simulink model "EV6_LUT_FourWheel_EV6Battery77p4kWh_PowerCorrected"  (R2024a)
settings: Solver=ode4  StartTime=0  StopTime=60  FixedStep=0.001  RelTol=1e-3
PreLoadFcn:
  | VSS_BICYCLE=Simulink.Variant('Dual=0');
  | VSS_DUAL=Simulink.Variant('Dual=1');
  | Dual=1;
  | load('DriveCycle2.mat')
PostLoadFcn:
  | if any(exist('dsrtsu_mdlpostloadfcn', 'file') ~= 0), dsrtsu_mdlpostloadfcn('Execute', bdroot); end
InitFcn:
  | , if any(exist('rtifpga_mdlclblib', 'file') ~= 0), rtifpga_mdlclblib('Init', bdroot); end,
  | , if any(exist('dsmpb_private', 'file') ~= 0), dsmpb_private('dsmpb_mdlclblib', 'Init', bdroot); end,
  | load('DriveCycle2.mat')
model workspace (MAT data in the model file):
  DiffRatio = 10.65
  EV6_2023_BattBranchCapacity_Ah = 55.5236728838
  EV6_2023_BattEnergy_kWh = 77.4
  EV6_2023_BattNominalVoltage_V = 697
  EV6_2023_BattNumCellsParallel = 2
  EV6_2023_BattNumCellsSeries = 192
  EV6_2023_BattOpenVoltCapBpts = [0 0.1 0.2 0.3 0.4 0.5 0.6 0.7 0.8 0.9 1]
  EV6_2023_BattOpenVoltTbl = [2.96762142548 3.40364281191 3.47417488548 3.54470541822 3.61523441014 3.68576186124 3.75628777151 3.82681214095 3.94527005036 4.07101207308 4.2120755254]
  EV6_2023_BattPackCapacity_Ah = 111.047345768
  EV6_2023_BattResistSocBpts = [0 0.2 0.4 0.6 0.8 1]
  EV6_2023_BattResistTbl = [0.0163620057716 0.0118174152018 0.00807187352333 0.00375663957972 0.00266904525531 0.00103635901355 0.0019014404175 0.0172368903217 0.0121226074867 0.00758541551769 0.00474065349228 0.00337561163613 ... (42 elements, 7x6)]
  EV6_2023_BattResistTempBpts = [243.1 253.1 263.1 273.1 283.1 298.1 313.1]
  EV6_2023_InitialPackOCV_V = 726.471714233
  EV6_2023_InitialSOC = 0.638878863672
  EV6_BattCellCapacity_Ah = 60.3
  EV6_BattInitialSOC = 0.638878863672
  EV6_BattOCV_Cell_V = [2.96762142548 3.40364281191 3.47417488548 3.54470541822 3.61523441014 3.68576186124 3.75628777151 3.82681214095 3.94527005036 4.07101207308 4.2120755254]
  EV6_BattOCV_SOC = [0 0.1 0.2 0.3 0.4 0.5 0.6 0.7 0.8 0.9 1]
  EV6_BattPackCapacity_Ah = 120.6
  EV6_BattParallelCells = 2
  EV6_BattResistanceSOC = [0 0.2 0.4 0.6 0.8 1]
  EV6_BattResistanceTable_Ohm = [0.0163620057716 0.0118174152018 0.00807187352333 0.00375663957972 0.00266904525531 0.00103635901355 0.0019014404175 0.0172368903217 0.0121226074867 0.00758541551769 0.00474065349228 0.00337561163613 ... (42 elements, 7x6)]
  EV6_BattResistanceTemp_K = [243.1 253.1 263.1 273.1 283.1 298.1 313.1]
  EV6_BattSeriesCells = 192
  EV6_FinalDriveRatio = 10.65
  EV6_TargetPackResistance_Ohm = 0.132763804608
  Gas = 0.383333333333
undefined symbols (not defined in the file): accel_bp_mps2, AccelCmd, ActTqLF_Nm_, ActTqLR_Nm_, ActTqRF_Nm_, ActTqRR_Nm_, BattChargeLimitMaxPwr, BattChargeLimitSocBpts, BattChargeLimitTbl, BattDischargeLimitSocBpts, BattDischargeLimitTbl, BattDischargeMaxPwr, BrakeMaxPrs, BrakeMaxTrq, ChassisDistCg2FrontAxle, ChassisDistCg2RearAxle, ChassisVehMass, CltchCmd, CoastDown, DecelCmd, DiscIntNeverNeededParam, EnvGravCnst, EnvPrs, EnvTemp, EV6_RegenTorqueGain, EV6_TractionTorqueGain, front_share_regen_3d, front_share_traction_3d, FuelSpecificGrav, GearCmd, h, InitStates, lgSw, limitedMCT, MCT, MtrEffSpdBpts, MtrEffTbl, MtrEffTrqBpts, MtrPwrMax, MtrTrqMax, out_1, pMCT, RealSimPara, Ref_speed, Ref_time, regen_torque_bp_Nm, speed_bp_kph, SteeringCmd, SupvsryCtrlRegenBrkCutOffTbl, SupvsryCtrlRegenSpdBpts, TestScnrioCycleNum, traction_torque_bp_Nm, US06, VEH
libraries: VSIGenLib x65, simulink x54, etargetslib x38, dsmpblib x24, vehdynlibtire x12, autolibshared x11, vehdynlibsuspension x7, vehdynlibtirecommon x7, autolibpowerinfoutils x6, autolibutils x5, autolibsharedcoupling x4, autolibmappedmotor x4
(part 6 of 19)

== system EV6_LUT_FourWheel_EV6Battery77p4kWh_PowerCorrected/Vehicle Under Test1/Vehicle/Battery/Battery ==
  note: Thermal model is needed to estimated battery temperature. Ambient temperture is assumed.
  Bus Creator1 : BusCreator  Inputs=1
  Bus Selector : BusSelector  OutputSignals=BattSoc
  Bus Selector1 : BusSelector  OutputSignals=Curr
  Bus Selector2 : BusSelector  OutputSignals=Curr
  Constant : Constant  Value=EnvTemp
  EV6 Speed Mode Power Correction : Subsystem
  Lithium Ion Battery Pack1 : Subsystem  AncestorBlock=autolibdatasheetbattery/Datasheet Battery  mask(Datasheet Battery){CapacityCtrl=Parameter, OutputVlt=Unfiltered, BattChargeMax=EV6_2023_BattBranchCapacity_Ah, Em=EV6_2023_BattOpenVoltTbl, CapLUTBp=EV6_2023_BattOpenVoltCapBpts, RInt=EV6_2023_BattResistTbl, BattTempBp=EV6_2023_BattResistTempBpts, CapSOCBp=EV6_2023_BattResistSocBpts, Ns=EV6_2023_BattNumCellsSeries, Np=EV6_2023_BattNumCellsParallel, BattCapInit=EV6_2023_InitialSOC*EV6_2023_BattBranchCapacity_Ah, Tc=1/1000, Vinit=EV6_2023_InitialPackOCV_V, RefBlkName='autolibdatasheetbattery/Datasheet Battery'}
      mask prompts: CapacityCtrl "autoblks:autoblkDatasheetBattery:blkPrm_CapacityCtrl"; OutputVlt "autoblks:autoblkDatasheetBattery:blkPrm_OutputVlt"; BattChargeMax "autoblks:autoblkDatasheetBattery:blkPrm_BattChargeMax"; Em "autoblks:autoblkDatasheetBattery:blkPrm_Em"; CapLUTBp "autoblks:autoblkDatasheetBattery:blkPrm_CapLUTBp"; RInt "autoblks:autoblkDatasheetBattery:blkPrm_RInt"; BattTempBp "autoblks:autoblkDatasheetBattery:blkPrm_BattTempBp"; CapSOCBp "autoblks:autoblkDatasheetBattery:blkPrm_CapSOCBp"; Ns "autoblks:autoblkDatasheetBattery:blkPrm_Ns"; Np "autoblks:autoblkDatasheetBattery:blkPrm_Np"; BattCapInit "autoblks:autoblkDatasheetBattery:blkPrm_BattCapInit"; Tc "autoblks:autoblkDatasheetBattery:blkPrm_Tc"; Vinit "autoblks:autoblkDatasheetBattery:blkPrm_Vinit"
      mask help: autoblks:autoblkDatasheetBattery:blkDesc
      mask init:
      | autoicon('autolibdatasheetbattery',gcb,'Initialization');
      mask Help: eval('autoblkshelp(''pbbatterydatasheet'')');
      mask TypeOptions CapacityCtrl: autoblks:autoblkDatasheetBattery:blkCmb_CapacityCtrlExternalInput | autoblks:autoblkDatasheetBattery:blkCmb_CapacityCtrlParameter
      mask TypeOptions OutputVlt: autoblks:autoblkDatasheetBattery:blkCmb_OutputVltFiltered | autoblks:autoblkDatasheetBattery:blkCmb_OutputVltUnfiltered
      mask DialogControl Container3 Prompt: autoblks:autoblkDatasheetBattery:blkDlg_Container3
      mask DialogControl CapacityCtrl Prompt: Initial battery capacity:
      mask DialogControl OutputVlt Prompt: Output battery voltage:
      mask DialogControl ParameterGroupVar Prompt: autoblks:autoblkDatasheetBattery:blkDlg_ParameterGroupVar
      mask DialogControl BattChargeMax Prompt: Rated capacity at nominal temperature, BattChargeMax [Ah]:
      mask DialogControl Em Prompt: Open circuit voltage table data, Em [V]:
      mask DialogControl CapLUTBp Prompt: Open circuit voltage breakpoints 1, CapLUTBp []:
      mask DialogControl RInt Prompt: Internal resistance table data, RInt [Ohms]:
      mask DialogControl BattTempBp Prompt: Battery temperature breakpoints 1, BattTempBp [K]:
      mask DialogControl CapSOCBp Prompt: Battery capacity breakpoints 2, CapSOCBp []:
      mask DialogControl Ns Prompt: Number of cells in series, Ns []:
      mask DialogControl Np Prompt: Number of cells in parallel, Np []:
      mask DialogControl BattCapInit Prompt: Initial battery capacity, BattCapInit [Ah]:
      mask DialogControl Tc Prompt: Output battery voltage time constant, Tc [s]:
      mask DialogControl Vinit Prompt: Output battery voltage initial value, Vinit [V]:
      mask Display:
      | IconInfo = autoicon('autolibdatasheetbattery', gcb, 'DrawCommands');
      | 
      | image(IconInfo.image, IconInfo.position);
      | 
      | for i = 1:numel(IconInfo.lconn)
      |     port_label('lconn', i, IconInfo.lconn{i})
      | end
      | 
      | for j = 1:numel(IconInfo.rconn)
      |     port_label('rconn', j, IconInfo.rconn{j})
      | end
      | 
      | for k = 1:numel(IconInfo.input)
      |     port_label('input', k, IconInfo.input{k})
      | end
      | 
      | for m = 1:numel(IconInfo.output)
      |     port_label('output', m, IconInfo.output{m})
      | end
  Log EV6 Base Power : ToWorkspace  VariableName=EV6BasePower_kW  SaveFormat=Timeseries  SampleTime=-1
  Log EV6 Current Correction : ToWorkspace  VariableName=EV6CurrentCorrection_A  SaveFormat=Timeseries  SampleTime=-1
  Log EV6 Power Correction : ToWorkspace  VariableName=EV6PowerCorrection_kW  SaveFormat=Timeseries  SampleTime=-1
  Sum : Sum  Inputs=|+++
  Two-Way Connection1 : TwoWayConnection
  Two-Way Connection2 : TwoWayConnection
  Batt : PMIOPort  Side=Right
  Batt1 : PMIOPort  Port=2  Side=Right
  BattSoc : Outport
  BattCurr : Outport  Port=2  Unit=A
  BattVolt : Outport  Port=3  Unit=V
  wires:
  Two-Way Connection1/1 -> Bus Selector2/1
  Lithium Ion Battery Pack1/1(Info) -> Bus Selector/1
  Bus Selector/1 -> BattSoc/1  "<BattSoc>"
  Constant/1 -> Lithium Ion Battery Pack1/2(BattTemp)
  Bus Creator1/1 -> Two-Way Connection2/1, Two-Way Connection1/1
  Lithium Ion Battery Pack1/2(BattVolt) -> Bus Creator1/1, BattVolt/1  "Volt"
  Two-Way Connection2/1 -> Bus Selector1/1
  Bus Selector1/1 -> Sum/2, EV6 Speed Mode Power Correction/3(RearCurrent_A)  "<Curr>"
  Bus Selector2/1 -> Sum/1, EV6 Speed Mode Power Correction/2(FrontCurrent_A)  "<Curr>"
  Sum/1 -> BattCurr/1, Lithium Ion Battery Pack1/1(BattCurr)
  [vehSpeedSim] -> EV6 Speed Mode Power Correction/1(VehicleSpeed_mps)
  EV6 Speed Mode Power Correction/1(CorrectionCurrent_A) -> Sum/3, Log EV6 Current Correction/1
  EV6 Speed Mode Power Correction/2(CorrectionPower_kW) -> Log EV6 Power Correction/1
  EV6 Speed Mode Power Correction/3(BasePower_kW) -> Log EV6 Base Power/1
  connections:
  Batt/RConn1 -- Two-Way Connection1/RConn1
  Batt1/RConn1 -- Two-Way Connection2/RConn1

== system EV6_LUT_FourWheel_EV6Battery77p4kWh_PowerCorrected/Vehicle Under Test1/Vehicle/Battery/Subsystem1 ==
  BattSoc : Inport
  BattCurr : Inport  Port=2
  BattVolt : Inport  Port=3
  Bus Creator : BusCreator  Inputs=3
  Batt : Outport
  wires:
  BattVolt/1 -> Bus Creator/3  "BattVolt"
  Bus Creator/1 -> Batt/1  "Batt"
  BattCurr/1 -> Bus Creator/2  "BattCurr"
  BattSoc/1 -> Bus Creator/1  "BattSoc"

== system EV6_LUT_FourWheel_EV6Battery77p4kWh_PowerCorrected/Vehicle Under Test1/Vehicle/Driver and Drive Cycle/Driver and PI with FF Control ==
  Vehicle_Spd_kph : Inport
  Vehicle_SpdDmd_kph : Inport  Port=2
  Bus Creator : BusCreator  Inputs=6
  Constant : Constant
  Memory1 : Memory
  Memory2 : Memory
  Scope1 : Scope  NumInputPorts=3
  Scope2 : Scope  NumInputPorts=3
  SpdSat : Saturate  UpperLimit=190  LowerLimit=-5
  Speed controller set : Subsystem
  km to miles : Gain  Gain=1/1.609344
  DriverBus : Outport
  wires:
  Speed controller set/2(BrakePedalCmd) -> Bus Creator/3, Scope2/2
  Speed controller set/1(AccelPedalCmd) -> Bus Creator/2, Scope2/1
  Memory2/1 -> Speed controller set/2(VehSpd)
  Memory1/1 -> SpdSat/1
  km to miles/1 -> Bus Creator/6  "RefSpd [mph]"
  Vehicle_Spd_kph/1 -> Memory2/1
  Bus Creator/1 -> DriverBus/1  "DriverBus"
  SpdSat/1 -> km to miles/1, Bus Creator/5, Speed controller set/1(RefSpd [km/hr])  "RefSpd [km/hr]"
  Constant/1 -> Bus Creator/1  "Drive"
  Vehicle_SpdDmd_kph/1 -> Memory1/1
  Speed controller set/3(BrakeSwitch) -> Bus Creator/4, Scope2/3

== system EV6_LUT_FourWheel_EV6Battery77p4kWh_PowerCorrected/Vehicle Under Test1/Vehicle/Driver and Drive Cycle/Get Cycle Clock Time ==
  Cycle Trigger : Inport
  Add1 : Sum  Inputs=+-
  Clock1 : Clock
  Clock2 : Clock
  Data Type Conversion : DataTypeConversion  OutDataTypeStr=double  SaturateOnIntegerOverflow=off  RndMeth=Floor
  Memory4 : Memory
  Switch : Switch  Criteria=u2 > Threshold  SaturateOnIntegerOverflow=off  InputSameDT=off
  tCycle : Outport
  wires:
  Data Type Conversion/1 -> Switch/2
  Cycle Trigger/1 -> Data Type Conversion/1
  Memory4/1 -> Switch/1
  Add1/1 -> tCycle/1  "tCycle"
  Clock2/1 -> Switch/3
  Clock1/1 -> Add1/1
  Switch/1 -> Memory4/1, Add1/2

== system EV6_LUT_FourWheel_EV6Battery77p4kWh_PowerCorrected/Vehicle Under Test1/Vehicle/Front Wheel Drive/Ideal Diff ==
  DrvShfTrq : Inport
  Omega : Inport  Port=2
  Add : Sum
  Add1 : Sum
  Bus Creator1 : BusCreator  Inputs=2
  Bus Creator2 : BusCreator  Inputs=2
  Bus Creator3 : BusCreator  Inputs=2
  Bus Creator4 : BusCreator  Inputs=4
  Bus to Vector : BusToVector
  Constant : Constant  Value=0
  Demux : Demux  Outputs=[2,2]
  Demux1 : Demux  Outputs=2
  Gain1 : Gain  Gain=0.5
  Gain2 : Gain  Gain=DiffRatio
  Gain3 : Gain  Gain=DiffRatio
  Gain4 : Gain  Gain=0.5
  Memory : Memory
  Memory1 : Memory
  Power Bus : Subsystem
  Terminator : Terminator
  Terminator1 : Terminator
  Vector Concatenate : Concatenate  NumInputs=4
  Diff : Outport  VectorParamsAs1DForOutWhenUnconnected=off
  AxlTrq : Outport  Port=2  VectorParamsAs1DForOutWhenUnconnected=off
  PropShaftSpd : Outport  Port=3  VectorParamsAs1DForOutWhenUnconnected=off
  wires:
  Demux1/2 -> [Axl2Spd], Add1/2
  Vector Concatenate/1 -> AxlTrq/1
  Gain4/1 -> [Axl1Trq], Add/1, Vector Concatenate/1, [Axl2Trq], Add/2, Vector Concatenate/2  "T_FL"
  DrvShfTrq/1 -> [DriveshftTrq], Bus to Vector/1
  [DriveshftTrq] -> Power Bus/1(DriveshftTrq), Bus Creator1/1  "DriveshftTrq"
  [Axl1Spd] -> Bus Creator2/2  "Axl1Spd"
  Demux/1 -> Demux1/1
  Add1/1 -> Gain1/1
  Bus Creator4/1 -> Diff/1
  Add/1 -> Terminator/1  "AxlTrqLump"
  [Axl2Trq] -> Bus Creator3/1  "Axl2Trq"
  Omega/1 -> Demux/1
  Memory/1 -> Gain3/1
  Bus to Vector/1 -> Memory/1
  Bus Creator3/1 -> Bus Creator4/3  "Axl2"
  Bus Creator2/1 -> Bus Creator4/2  "Axl1"
  Bus Creator1/1 -> Bus Creator4/1  "Driveshft"
  [DriveshftSpd] -> Bus Creator1/2, Power Bus/2(Speed)  "Speed"
  Gain2/1 -> Memory1/1  "Spd"
  Constant/1 -> Vector Concatenate/4, Vector Concatenate/3  "T_RR"
  Demux1/1 -> [Axl1Spd], Add1/1
  Memory1/1 -> PropShaftSpd/1, [DriveshftSpd]
  Gain3/1 -> Gain4/1
  [Axl1Trq] -> Bus Creator2/1  "Axl1Trq"
  Power Bus/1(PwrInfo) -> Bus Creator4/4
  Gain1/1 -> Gain2/1
  [Axl2Spd] -> Bus Creator3/2  "Axl2Spd"
  Demux/2 -> Terminator1/1

== system EV6_LUT_FourWheel_EV6Battery77p4kWh_PowerCorrected/Vehicle Under Test1/Vehicle/Front Wheel Drive/Ideal Diff AWD ==
  note: FrontAxlTrq_Sim
  DrvShfTrq : Inport
  Omega : Inport  Port=2
  Add : Sum
  Add1 : Sum
  Add2 : Sum  Commented=on
  Bus Creator1 : BusCreator  Inputs=2
  Bus Creator2 : BusCreator  Inputs=2
  Bus Creator3 : BusCreator  Inputs=2
  Bus Creator4 : BusCreator  Inputs=4
  Bus to Vector : BusToVector
  Demux : Demux  Outputs=[2,2]
  Demux1 : Demux  Outputs=2
  Demux2 : Demux  Commented=on  Outputs=2
  Demux3 : Demux  Commented=on  Outputs=2
  From Workspace2 : FromWorkspace  Commented=on  VariableName=ts_WheelSpd_Front
  Gain : Gain  Commented=on  Gain=pi/30
  Gain1 : Gain  Gain=0.5
  Gain2 : Gain  Gain=EV6_FinalDriveRatio
  Gain3 : Gain  Gain=EV6_FinalDriveRatio
  Gain4 : Gain  Gain=0.5
  Gain5 : Gain  Commented=on  Gain=0.5
  Gain6 : Gain  Commented=on  Gain=DiffRatio
  Gain7 : Gain  Commented=on  Gain=pi/30
  Goto10 : Goto  Commented=on  GotoTag=DriveshftSpd
  Goto8 : Goto  Commented=on  GotoTag=Axl2Spd
  Goto9 : Goto  Commented=on  GotoTag=Axl1Spd
  Memory : Memory
  Memory1 : Memory
  Memory2 : Memory  Commented=on
  Power Bus : Subsystem
  Scope : Scope
  Scope1 : Scope
  Scope2 : Scope
  Terminator : Terminator
  Terminator1 : Terminator  Commented=on
  Terminator2 : Terminator
  Vector Concatenate : Concatenate
  Diff : Outport  VectorParamsAs1DForOutWhenUnconnected=off
  AxlTrq : Outport  Port=2  VectorParamsAs1DForOutWhenUnconnected=off
  PropShaftSpd : Outport  Port=3  VectorParamsAs1DForOutWhenUnconnected=off
  wires:
  Gain7/1 -> Goto8/1, Add2/2
  Gain/1 -> Add2/1, Goto9/1
  Add2/1 -> Gain5/1
  Memory2/1 -> Terminator1/1, Goto10/1
  Gain6/1 -> Memory2/1  "Spd"
  Gain5/1 -> Gain6/1
  DrvShfTrq/1 -> Bus to Vector/1, [DriveshftTrq]
  Power Bus/1(PwrInfo) -> Bus Creator4/4
  Demux1/2 -> Add1/2, [Axl2Spd]
  Gain4/1 -> [Axl1Trq], Add/1, Vector Concatenate/1, [Axl2Trq], Add/2, Vector Concatenate/2, Scope1/1  "T_FL"
  Demux/2 -> Terminator2/1
  Vector Concatenate/1 -> AxlTrq/1, Scope2/1
  Gain1/1 -> Gain2/1
  Gain3/1 -> Gain4/1, Scope/1
  [Axl1Trq] -> Bus Creator2/1  "Axl1Trq"
  Bus to Vector/1 -> Memory/1
  Gain2/1 -> Memory1/1  "Spd"
  Memory/1 -> Gain3/1
  Bus Creator2/1 -> Bus Creator4/2  "Axl1"
  Memory1/1 -> PropShaftSpd/1, [DriveshftSpd]
  Demux1/1 -> [Axl1Spd], Add1/1
  [DriveshftSpd] -> Bus Creator1/2  "Speed"
  Bus Creator4/1 -> Diff/1
  [Axl2Spd] -> Bus Creator3/2  "Axl2Spd"
  Bus Creator1/1 -> Bus Creator4/1  "Driveshft"
  Add/1 -> Terminator/1  "AxlTrqLump"
  [Axl1Spd] -> Bus Creator2/2  "Axl1Spd"
  [Axl2Trq] -> Bus Creator3/1  "Axl2Trq"
  Demux/1 -> Demux1/1
  Bus Creator3/1 -> Bus Creator4/3  "Axl2"
  [DriveshftTrq] -> Bus Creator1/1  "DriveshftTrq"
  Add1/1 -> Gain1/1
  [DriveshftTrq] -> Power Bus/1(DriveshftTrq)  "DriveshftTrq"
  [DriveshftSpd] -> Power Bus/2(Speed)  "Speed"
  Omega/1 -> Demux/1
  From Workspace2/1 -> Demux3/1
  Demux3/1 -> Gain/1
  Demux3/2 -> Gain7/1

== system EV6_LUT_FourWheel_EV6Battery77p4kWh_PowerCorrected/Vehicle Under Test1/Vehicle/Front Wheel Drive/Real Diff ==
  DrvShfTrq : Inport
  Omega : Inport  Port=2
  Bus Creator1 : BusCreator  Inputs=2
  Bus Creator2 : BusCreator  Inputs=2
  Bus Creator3 : BusCreator  Inputs=2
  Bus Creator4 : BusCreator  Inputs=4
  Constant : Constant  Value=0
  Demux : Demux  Outputs=[2,2]
  Demux1 : Demux  Outputs=2
  DiffPress : Constant  Value=0
  Limited Slip Differential : autolibshareddiff/Limited Slip Differential  DiffEffModelPopup=Constant  InterpMethod=Linear point-slope  extTamb=off  shaftSwitchMask=To the left of center-line  Ndiff=7.05  Jd=0.025  bd=1e-3  Jw1=0.01  bw1=1e-3  Jw2=0.01  bw2=1e-3  omegaw1o=0  omegaw2o=0  eta=0.98  eta_tbl=reshape([0.64 0.76 0.8 0.81 0.83 0.84 0.84 0.56 0.73 0.78 0.8 0.83 0.84 0.84 0.54 0.71 0.77 0.8 0.82 0.84 0.84 0.53 0.71 0.77 0.8 0.83 0.84 0.84 0.51 0.71 0.77 0.8 0.83 0.84 0.85 0.52 0.7 0.77 0.8 0.83 0.84 0.85 0.51 0.71 0.76 0.79 0.83 0.84 0.85 0.5 0.69 0.76 0.79 0.82 0.84 0.85 0.45 0.68 0.75 0.78 0.82 0.84 0.85 0.43 0.67 0.74 0.78 0.81 0.83 0.84 0.38 0.63 0.71 0.75 0.8 0.82 0.83 0.81 0.86 0.88 0.89 0.89 0.89 0.9 0.77 0.85 0.87 0.88 0.89 0.9 0.9 0.72 0.82 0.86 0.87 0.88 0.89 0.9 0.68 0.8 0.84 0.86 0.88 0.89 0.89 0.67 0.8 0.84 0.86 0.88 0.89 0.9 0.67 0.8 0.84 0.86 0.88 0.89 0.9 0.65 0.8 0.84 0.86 0.88 0.89 0.9 0.64 0.79 0.83 0.86 0.88 0.89 0.9 0.63 0.78 0.83 0.86 0.88 0.89 0.9 0.59 0.76 0.82 0.85 0.87 0.89 0.9 0.53 0.73 0.8 0.83 0.86 0.88 0.89], 7, 11, 2)  Trq_bpts=[25, 50, 75, 100, 150, 200, 250]  omega_bpts=[52.4 78.5 105 131 157 183 209 262 314 419 524]  Temp_bpts=[290 358]  Tamb=297.15  couplingType=Pre-loaded ideal clutch  Ndisks=8  Reff=.08  Fc=1000  muc=[.16 0.13 0.115 0.11 0.105 0.1025 0.10125 .10125]  dw=[0 10 20 40 60 80 100 1000]  Tdw=[-100, -90, -50, -5, 0, 5, 50, 90, 100]  dwT=[-200, -175, -100, - 50, 0, 50, 100, 175, 200]  TTin=[-200 -175 -100 - 50 0 50 100 175 200]  Tin=[-200 -175 -100 - 50 0 50 100 175 200]  tauC=.04  IdealInterpMethod=Linear point-slope  IdealExtrapMethod=Linear  TdwInterpMethod=Flat  TdwExtrapMethod=Clip  TTinInterpMethod=Flat  TTinExtrapMethod=Clip  maxAbsSpd=5e3  aMode=2
      settings: LibrarySourceBlock=vdynlib/Powertrain/Drivetrain/Final Drive Unit/Limited Slip Differential
  Power Bus : Subsystem
  Terminator : Terminator
  Terminator1 : Terminator
  Terminator3 : Terminator
  Torsional Compliance1 : autolibsharedcoupling/Torsional Compliance  port_config=Simulink  extInfo=off  k=10000  b=400  theta_o=0  domega_o=0  omega_c=300  blkID=0  aMode=2
      settings: LibrarySourceBlock=vdynlib/Powertrain/Drivetrain/Couplings/Torsional Compliance
  Torsional Compliance2 : autolibsharedcoupling/Torsional Compliance  port_config=Simulink  extInfo=off  k=10000  b=400  theta_o=0  domega_o=0  omega_c=300  blkID=0  aMode=2
      settings: LibrarySourceBlock=vdynlib/Powertrain/Drivetrain/Couplings/Torsional Compliance
  Vector Concatenate : Concatenate  NumInputs=4
  Vector Concatenate1 : Concatenate  NumInputs=4
  Diff : Outport  VectorParamsAs1DForOutWhenUnconnected=off
  AxlTrq : Outport  Port=2  VectorParamsAs1DForOutWhenUnconnected=off
  PropShaftSpd : Outport  Port=3  VectorParamsAs1DForOutWhenUnconnected=off
  wires:
  Limited Slip Differential/3 -> [Axl1Spd], Torsional Compliance2/1
  Demux1/1 -> Torsional Compliance2/2
  Limited Slip Differential/1 -> Terminator/1
  DrvShfTrq/1 -> [DriveshftTrq], Limited Slip Differential/1
  Limited Slip Differential/4 -> [Axl2Spd], Torsional Compliance1/1
  Demux1/2 -> Torsional Compliance1/2
  Demux/1 -> Demux1/1
  Torsional Compliance1/1 -> Limited Slip Differential/3
  Torsional Compliance2/1 -> Limited Slip Differential/2
  Demux/2 -> Terminator1/1
  Constant/1 -> Vector Concatenate/4, Vector Concatenate/3  "T_RR"
  Torsional Compliance1/2 -> [Axl2Trq], Vector Concatenate/2  "T_FR"
  Torsional Compliance2/2 -> [Axl1Trq], Vector Concatenate/1  "T_FL"
  Omega/1 -> Demux/1
  Vector Concatenate/1 -> AxlTrq/1
  Vector Concatenate1/1 -> Terminator3/1
  DiffPress/1 -> Vector Concatenate1/4, Vector Concatenate1/3, Vector Concatenate1/1, Vector Concatenate1/2
  [DriveshftTrq] -> Power Bus/1(DriveshftTrq), Bus Creator1/1  "DriveshftTrq"
  [Axl1Spd] -> Bus Creator2/2  "Axl1Spd"
  [Axl2Trq] -> Bus Creator3/1  "Axl2Trq"
  Bus Creator4/1 -> Diff/1
  [Axl2Spd] -> Bus Creator3/2  "Axl2Spd"
  [DriveshftSpd] -> Bus Creator1/2, Power Bus/2(Speed)  "Speed"
  Bus Creator1/1 -> Bus Creator4/1  "Driveshft"
  [Axl1Trq] -> Bus Creator2/1  "Axl1Trq"
  Power Bus/1(PwrInfo) -> Bus Creator4/4
  Bus Creator2/1 -> Bus Creator4/2  "Axl1"
  Bus Creator3/1 -> Bus Creator4/3  "Axl2"
  Limited Slip Differential/2 -> [DriveshftSpd], PropShaftSpd/1

== system EV6_LUT_FourWheel_EV6Battery77p4kWh_PowerCorrected/Vehicle Under Test1/Vehicle/Powertrain Supervisory Controller /Engine Torque Command ==
  AccelCmdIn : Inport
  DecelCmdIn : Inport  Port=2
  DriverGearCmdIn : Inport  Port=3
  VehSpd : Inport  Port=4
  BattSoc : Inport  Port=5
  MtrSpd : Inport  Port=6
  VehAcc : Inport  Port=7
  Accel Pedal to Traction Wheel Torque Request1 : Subsystem
  Accelerator Command Display : Display
  Battery Management System : Subsystem
  Brake Command Display : Display
  EV6 Regen Calibration Gain : Gain  Gain=EV6_RegenTorqueGain
  EV6 Torque Distribution : Subsystem
  EV6 Traction Calibration Gain : Gain  Gain=EV6_TractionTorqueGain
  Final MtrTrqCmd Display (N*m) : Display
  From : From  Commented=on  GotoTag=MotSpd
  From Workspace : FromWorkspace  VariableName=ts_VehSpd
  Front MtrTrqCmd Display (N*m) : Display
  Front Torque Share Display : Display
  Front share : ToWorkspace  VariableName=FrontShare_log  SaveFormat=Timeseries  SampleTime=-1
  Front torque command : ToWorkspace  VariableName=FrontMtrTrqCmd_log  SaveFormat=Timeseries  SampleTime=-1
  Gain : Gain  Gain=2.2369
  Gain1 : Gain  Gain=3.6
  Gain2 : Gain  Gain=2.23694
  Motor Torque Arbitration and Power Management : Subsystem
  Original final torque : ToWorkspace  VariableName=TotalMtrTrqCmd_log  SaveFormat=Timeseries  SampleTime=-1
  Rear MtrTrqCmd Display (N*m) : Display
  Rear Torque Share Display : Display
  Rear share : ToWorkspace  VariableName=RearShare_log  SaveFormat=Timeseries  SampleTime=-1
  Rear torque command : ToWorkspace  VariableName=RearMtrTrqCmd_log  SaveFormat=Timeseries  SampleTime=-1
  Scope : Scope
  Scope1 : Scope
  Series Regen Braking : Subsystem  InitFcn=%[~]=autosharedicon('autolibutils',gcb,0);  VariantControl=Variant
  Terminator : Terminator
  VehSpd inside ETC : Display
  "Vehicle Speed Display(m/s) " : Display
  MtrTrqCmd : Outport
  AccelCmd : Outport  Port=2
  BrkCmd : Outport  Port=3
  DriverGearCmd : Outport  Port=4
  FrontMtrTrqCmd : Outport  Port=5
  RearMtrTrqCmd : Outport  Port=6
  wires:
  Accel Pedal to Traction Wheel Torque Request1/1(TrqCmd) -> EV6 Traction Calibration Gain/1  "MotTrqCmdTrac_PreArbitration"
  Motor Torque Arbitration and Power Management/1(MotTrqCmdFinal) -> EV6 Torque Distribution/3(MtrTrqCmd), Final MtrTrqCmd Display (N*m)/1, MtrTrqCmd/1, Original final torque/1  "MotTrqCmd_Final"
  [MotSpd] -> Motor Torque Arbitration and Power Management/5(MotSpd)  "MotSpd_ETC_radps"
  Series Regen Braking/1(" MotTrqCmdRegen") -> EV6 Regen Calibration Gain/1  "MotTrqCmdRegen_PreArbitration"
  Battery Management System/2(BattPwrChrgLmt) -> Motor Torque Arbitration and Power Management/4("BattPwrChrgLmt ")  "BattPwrChrgLmt"
  Series Regen Braking/2(" BrkCmd") -> Scope/1, BrkCmd/1  "BrkCmd"
  Battery Management System/1(BattPwrDischrgLmt) -> Motor Torque Arbitration and Power Management/3(BattPwrDisChrgLmt)  "BattPwrDischrgLmt"
  BattSoc/1 -> Series Regen Braking/1(BattSoc), Battery Management System/1(SOC)  "SOC"
  AccelCmdIn/1 -> Accelerator Command Display/1, [AccelPdl], Accel Pedal to Traction Wheel Torque Request1/1(AccelPdl), AccelCmd/1
  MtrSpd/1 -> [MotSpd], Series Regen Braking/3(MotSpd)  "MotSpd"
  [AccelPdl] -> Motor Torque Arbitration and Power Management/2(AccelPdl)
  DriverGearCmdIn/1 -> DriverGearCmd/1
  DecelCmdIn/1 -> Brake Command Display/1, Series Regen Braking/4("DecelCmd "), Scope1/1  "DecelPdl"
  VehSpd/1 -> VehSpd inside ETC/1, Gain1/1, [VehSpd], Series Regen Braking/2(VehSpd), Gain2/1  "VehSpd"
  VehAcc/1 -> EV6 Torque Distribution/1(Accel_mps2)  "VehAcc_LUT_Input_mps2"
  Gain1/1 -> EV6 Torque Distribution/2(Speed_kph)
  EV6 Torque Distribution/4(RearMtrTrqCmd) -> RearMtrTrqCmd/1, Rear torque command/1, Rear MtrTrqCmd Display (N*m)/1
  EV6 Torque Distribution/2(RearShare) -> Rear share/1, Rear Torque Share Display/1  "RearShare"
  EV6 Torque Distribution/1(FrontShare) -> Front share/1, Front Torque Share Display/1  "FrontShare"
  EV6 Torque Distribution/3(FrontMtrTrqCmd) -> FrontMtrTrqCmd/1, Front torque command/1, Front MtrTrqCmd Display (N*m)/1
  Gain2/1 -> Accel Pedal to Traction Wheel Torque Request1/2(VehSpd_mph)
  EV6 Traction Calibration Gain/1 -> Motor Torque Arbitration and Power Management/1(MotTrqCmdTrac)  "MotTrqCmdTrac_Calibrated"
  EV6 Regen Calibration Gain/1 -> Motor Torque Arbitration and Power Management/6(MotTrqCmdRegen)  "MotTrqCmdRegen_Calibrated"

== system EV6_LUT_FourWheel_EV6Battery77p4kWh_PowerCorrected/Vehicle Under Test1/Vehicle/Powertrain Supervisory Controller /Subsystem1 ==
  MtrTrqCmd : Inport
  AccelCmd : Inport  Port=2
  BrkCmd : Inport  Port=3
  DriverGearCmd : Inport  Port=4
  SteeringCmd : Inport  Port=5
  Bus Creator : BusCreator  Inputs=5  OutDataTypeStr=Bus: SupvsryCtrlBus  NonVirtualBus=on
  SupvsryCtrl : Outport
  wires:
  SteeringCmd/1 -> Bus Creator/5  "SteeringCmd"
  DriverGearCmd/1 -> Bus Creator/4  "DriverGearCmd"
  BrkCmd/1 -> Bus Creator/3  "BrkCmd"
  AccelCmd/1 -> Bus Creator/2  "AccelCmd"
  Bus Creator/1 -> SupvsryCtrl/1  "SupvsryCtrl"
  MtrTrqCmd/1 -> Bus Creator/1  "MtrTrqCmd"

== system EV6_LUT_FourWheel_EV6Battery77p4kWh_PowerCorrected/Vehicle Under Test1/Vehicle/Powertrain Supervisory Controller /Subsystem4 ==
  Driver : Inport
  Chassis : Inport  Port=2
  Batt : Inport  Port=3
  Mtr : Inport  Port=4
  Bus Selector : BusSelector  OutputSignals=AccelCmd,DecelCmd,GearCmd
  Bus Selector1 : BusSelector  OutputSignals=VehSpd
  Bus Selector2 : BusSelector  OutputSignals=BattSoc
  Bus Selector3 : BusSelector  OutputSignals=MtrSpd
  VehSpd from Chassis : Display
  AccelCmd : Outport  VectorParamsAs1DForOutWhenUnconnected=off
  DecelCmd : Outport  Port=2  VectorParamsAs1DForOutWhenUnconnected=off
  DriverGearCmd : Outport  Port=3  VectorParamsAs1DForOutWhenUnconnected=off
  VehSpd : Outport  Port=4  VectorParamsAs1DForOutWhenUnconnected=off
  BattSoc : Outport  Port=5  VectorParamsAs1DForOutWhenUnconnected=off
  MtrSpd : Outport  Port=6  VectorParamsAs1DForOutWhenUnconnected=off
  wires:
  Bus Selector3/1 -> MtrSpd/1  "<MtrSpd>"
  Mtr/1 -> Bus Selector3/1
  Bus Selector2/1 -> BattSoc/1  "<BattSoc>"
  Batt/1 -> Bus Selector2/1
  Bus Selector/2 -> DecelCmd/1  "<DecelCmd>"
  Bus Selector1/1 -> VehSpd from Chassis/1, VehSpd/1  "<VehSpd>"
  Chassis/1 -> Bus Selector1/1
  Bus Selector/3 -> DriverGearCmd/1  "<GearCmd>"
  Bus Selector/1 -> AccelCmd/1  "<AccelCmd>"
  Driver/1 -> Bus Selector/1

== system EV6_LUT_FourWheel_EV6Battery77p4kWh_PowerCorrected/Vehicle Under Test1/Vehicle/Rear Wheel Drive/Ideal Diff ==
  DrvShfTrq : Inport
  Omega : Inport  Port=2
  Add : Sum
  Add1 : Sum
  Bus Creator1 : BusCreator  Inputs=2
  Bus Creator2 : BusCreator  Inputs=2
  Bus Creator3 : BusCreator  Inputs=2
  Bus Creator4 : BusCreator  Inputs=4
  Bus to Vector : BusToVector
  Constant : Constant  Value=0
  Demux : Demux  Outputs=[2,2]
  Demux1 : Demux  Outputs=2
  Gain1 : Gain  Gain=0.5
  Gain2 : Gain  Gain=DiffRatio
  Gain3 : Gain  Gain=DiffRatio
  Gain4 : Gain  Gain=0.5
  Memory : Memory
  Memory1 : Memory
  Power Bus : Subsystem
  Terminator : Terminator
  Terminator1 : Terminator
  Vector Concatenate : Concatenate  NumInputs=4
  Diff : Outport  VectorParamsAs1DForOutWhenUnconnected=off
  AxlTrq : Outport  Port=2  VectorParamsAs1DForOutWhenUnconnected=off
  PropShaftSpd : Outport  Port=3  VectorParamsAs1DForOutWhenUnconnected=off
  wires:
  Demux/2 -> Terminator1/1
  [Axl2Spd] -> Bus Creator3/2  "Axl2Spd"
  Gain1/1 -> Gain2/1
  Power Bus/1(PwrInfo) -> Bus Creator4/4
  [Axl1Trq] -> Bus Creator2/1  "Axl1Trq"
  Gain3/1 -> Gain4/1
  Memory1/1 -> [DriveshftSpd], PropShaftSpd/1
  Demux1/1 -> Add1/1, [Axl1Spd]
  Constant/1 -> Vector Concatenate/3, Vector Concatenate/4  "T_RR"
  Gain2/1 -> Memory1/1  "Spd"
  [DriveshftSpd] -> Power Bus/2(Speed), Bus Creator1/2  "Speed"
  Bus Creator1/1 -> Bus Creator4/1  "Driveshft"
  Bus Creator2/1 -> Bus Creator4/2  "Axl1"
  Bus Creator3/1 -> Bus Creator4/3  "Axl2"
  Bus to Vector/1 -> Memory/1
  Memory/1 -> Gain3/1
  Omega/1 -> Demux/1
  [Axl2Trq] -> Bus Creator3/1  "Axl2Trq"
  Add/1 -> Terminator/1  "AxlTrqLump"
  Bus Creator4/1 -> Diff/1
  Add1/1 -> Gain1/1
  Demux/1 -> Demux1/1
  [Axl1Spd] -> Bus Creator2/2  "Axl1Spd"
  [DriveshftTrq] -> Bus Creator1/1, Power Bus/1(DriveshftTrq)  "DriveshftTrq"
  DrvShfTrq/1 -> Bus to Vector/1, [DriveshftTrq]
  Gain4/1 -> Vector Concatenate/2, Add/2, [Axl2Trq], Vector Concatenate/1, Add/1, [Axl1Trq]  "T_FL"
  Vector Concatenate/1 -> AxlTrq/1
  Demux1/2 -> Add1/2, [Axl2Spd]

== system EV6_LUT_FourWheel_EV6Battery77p4kWh_PowerCorrected/Vehicle Under Test1/Vehicle/Rear Wheel Drive/Ideal Diff AWD ==
  note: RearAxlTrq_Sim
  DrvShfTrq : Inport
  Omega : Inport  Port=2
  Add : Sum  Commented=on
  Add1 : Sum  Inputs=++++
  Add2 : Sum  Commented=on
  Bus Creator1 : BusCreator  Inputs=2
  Bus Creator2 : BusCreator  Inputs=2
  Bus Creator3 : BusCreator  Inputs=2
  Bus Creator4 : BusCreator  Inputs=4
  Bus to Vector : BusToVector
  Demux : Demux  Outputs=[2,2]
  Demux1 : Demux  Commented=on  Outputs=2
  Demux2 : Demux  Outputs=2
  Demux3 : Demux  Commented=on  Outputs=2
  From Workspace4 : FromWorkspace  Commented=on  VariableName=ts_WheelSpd_Rear
  Gain1 : Gain  Gain=0.5
  Gain2 : Gain  Gain=EV6_FinalDriveRatio
  Gain3 : Gain  Gain=EV6_FinalDriveRatio
  Gain4 : Gain  Gain=0.5
  Gain5 : Gain  Commented=on  Gain=0.25
  Gain6 : Gain  Commented=on  Gain=10.4
  Gain7 : Gain  Commented=on  Gain=DiffRatio
  Gain8 : Gain  Commented=on  Gain=pi/30
  Gain9 : Gain  Commented=on  Gain=pi/30
  Goto10 : Goto  Commented=on  GotoTag=DriveshftSpd
  Goto8 : Goto  Commented=on  GotoTag=Axl2Spd
  Goto9 : Goto  Commented=on  GotoTag=Axl1Spd
  Memory : Memory
  Memory1 : Memory
  Memory2 : Memory  Commented=on
  Power Bus : Subsystem
  Scope : Scope
  Scope1 : Scope
  Scope2 : Scope
  Terminator : Terminator  Commented=on
  Terminator1 : Terminator
  Terminator2 : Terminator
  Vector Concatenate : Concatenate
  Diff : Outport  VectorParamsAs1DForOutWhenUnconnected=off
  AxlTrq : Outport  Port=2  VectorParamsAs1DForOutWhenUnconnected=off
  PropShaftSpd : Outport  Port=3  VectorParamsAs1DForOutWhenUnconnected=off
  wires:
  [DriveshftSpd] -> Power Bus/2(Speed)  "Speed"
  [DriveshftTrq] -> Power Bus/1(DriveshftTrq)  "DriveshftTrq"
  Demux2/2 -> [Axl2Spd], Add1/4
  Demux2/1 -> [Axl1Spd], Add1/3
  Add1/1 -> Gain1/1
  [DriveshftTrq] -> Bus Creator1/1  "DriveshftTrq"
  Bus Creator3/1 -> Bus Creator4/3  "Axl2"
  Demux/1 -> Terminator2/1
  [Axl2Trq] -> Bus Creator3/1  "Axl2Trq"
  [Axl1Spd] -> Bus Creator2/2  "Axl1Spd"
  Add/1 -> Terminator/1  "AxlTrqLump"
  Bus Creator1/1 -> Bus Creator4/1  "Driveshft"
  [Axl2Spd] -> Bus Creator3/2  "Axl2Spd"
  Bus Creator4/1 -> Diff/1
  [DriveshftSpd] -> Bus Creator1/2  "Speed"
  Memory1/1 -> PropShaftSpd/1, [DriveshftSpd]
  Bus Creator2/1 -> Bus Creator4/2  "Axl1"
  Memory/1 -> Gain3/1
  Gain2/1 -> Memory1/1  "Spd"
  Bus to Vector/1 -> Memory/1
  [Axl1Trq] -> Bus Creator2/1  "Axl1Trq"
  Gain3/1 -> Scope/1, Gain4/1
  Gain1/1 -> Gain2/1
  Vector Concatenate/1 -> Scope2/1, AxlTrq/1
  Demux/2 -> Demux2/1
  Gain4/1 -> Scope1/1, [Axl4Trq], Vector Concatenate/2, [Axl3Trq], Vector Concatenate/1  "T_RR"
  Power Bus/1(PwrInfo) -> Bus Creator4/4
  DrvShfTrq/1 -> [DriveshftTrq], Bus to Vector/1
  Gain5/1 -> Gain6/1
  Gain6/1 -> Memory2/1  "Spd"
  Memory2/1 -> Terminator1/1, Goto10/1
  Add2/1 -> Gain5/1
  Gain8/1 -> Goto9/1, Add2/1, Goto8/1
  Gain9/1 -> Add2/2
  Omega/1 -> Demux/1
  From Workspace4/1 -> Demux3/1
  Demux3/1 -> Gain8/1
  Demux3/2 -> Gain9/1

== system EV6_LUT_FourWheel_EV6Battery77p4kWh_PowerCorrected/Vehicle Under Test1/Vehicle/Rear Wheel Drive/Real Diff ==
  DrvShfTrq : Inport
  Omega : Inport  Port=2
  Bus Creator1 : BusCreator  Inputs=2
  Bus Creator2 : BusCreator  Inputs=2
  Bus Creator3 : BusCreator  Inputs=2
  Bus Creator4 : BusCreator  Inputs=4
  Constant : Constant  Value=0
  Demux : Demux  Outputs=[2,2]
  Demux1 : Demux  Outputs=2
  DiffPress : Constant  Value=0
  Limited Slip Differential : autolibshareddiff/Limited Slip Differential  DiffEffModelPopup=Constant  InterpMethod=Linear point-slope  extTamb=off  shaftSwitchMask=To the left of center-line  Ndiff=7.05  Jd=0.025  bd=1e-3  Jw1=0.01  bw1=1e-3  Jw2=0.01  bw2=1e-3  omegaw1o=0  omegaw2o=0  eta=0.98  eta_tbl=reshape([0.64 0.76 0.8 0.81 0.83 0.84 0.84 0.56 0.73 0.78 0.8 0.83 0.84 0.84 0.54 0.71 0.77 0.8 0.82 0.84 0.84 0.53 0.71 0.77 0.8 0.83 0.84 0.84 0.51 0.71 0.77 0.8 0.83 0.84 0.85 0.52 0.7 0.77 0.8 0.83 0.84 0.85 0.51 0.71 0.76 0.79 0.83 0.84 0.85 0.5 0.69 0.76 0.79 0.82 0.84 0.85 0.45 0.68 0.75 0.78 0.82 0.84 0.85 0.43 0.67 0.74 0.78 0.81 0.83 0.84 0.38 0.63 0.71 0.75 0.8 0.82 0.83 0.81 0.86 0.88 0.89 0.89 0.89 0.9 0.77 0.85 0.87 0.88 0.89 0.9 0.9 0.72 0.82 0.86 0.87 0.88 0.89 0.9 0.68 0.8 0.84 0.86 0.88 0.89 0.89 0.67 0.8 0.84 0.86 0.88 0.89 0.9 0.67 0.8 0.84 0.86 0.88 0.89 0.9 0.65 0.8 0.84 0.86 0.88 0.89 0.9 0.64 0.79 0.83 0.86 0.88 0.89 0.9 0.63 0.78 0.83 0.86 0.88 0.89 0.9 0.59 0.76 0.82 0.85 0.87 0.89 0.9 0.53 0.73 0.8 0.83 0.86 0.88 0.89], 7, 11, 2)  Trq_bpts=[25, 50, 75, 100, 150, 200, 250]  omega_bpts=[52.4 78.5 105 131 157 183 209 262 314 419 524]  Temp_bpts=[290 358]  Tamb=297.15  couplingType=Pre-loaded ideal clutch  Ndisks=8  Reff=.08  Fc=1000  muc=[.16 0.13 0.115 0.11 0.105 0.1025 0.10125 .10125]  dw=[0 10 20 40 60 80 100 1000]  Tdw=[-100, -90, -50, -5, 0, 5, 50, 90, 100]  dwT=[-200, -175, -100, - 50, 0, 50, 100, 175, 200]  TTin=[-200 -175 -100 - 50 0 50 100 175 200]  Tin=[-200 -175 -100 - 50 0 50 100 175 200]  tauC=.04  IdealInterpMethod=Linear point-slope  IdealExtrapMethod=Linear  TdwInterpMethod=Flat  TdwExtrapMethod=Clip  TTinInterpMethod=Flat  TTinExtrapMethod=Clip  maxAbsSpd=5e3  aMode=2
      settings: LibrarySourceBlock=vdynlib/Powertrain/Drivetrain/Final Drive Unit/Limited Slip Differential
  Power Bus : Subsystem
  Terminator : Terminator
  Terminator1 : Terminator
  Terminator3 : Terminator
  Torsional Compliance1 : autolibsharedcoupling/Torsional Compliance  port_config=Simulink  extInfo=off  k=10000  b=400  theta_o=0  domega_o=0  omega_c=300  blkID=0  aMode=2
      settings: LibrarySourceBlock=vdynlib/Powertrain/Drivetrain/Couplings/Torsional Compliance
  Torsional Compliance2 : autolibsharedcoupling/Torsional Compliance  port_config=Simulink  extInfo=off  k=10000  b=400  theta_o=0  domega_o=0  omega_c=300  blkID=0  aMode=2
      settings: LibrarySourceBlock=vdynlib/Powertrain/Drivetrain/Couplings/Torsional Compliance
  Vector Concatenate : Concatenate  NumInputs=4
  Vector Concatenate1 : Concatenate  NumInputs=4
  Diff : Outport  VectorParamsAs1DForOutWhenUnconnected=off
  AxlTrq : Outport  Port=2  VectorParamsAs1DForOutWhenUnconnected=off
  PropShaftSpd : Outport  Port=3  VectorParamsAs1DForOutWhenUnconnected=off
  wires:
  Limited Slip Differential/2 -> PropShaftSpd/1, [DriveshftSpd]
  Bus Creator3/1 -> Bus Creator4/3  "Axl2"
  Bus Creator2/1 -> Bus Creator4/2  "Axl1"
  Power Bus/1(PwrInfo) -> Bus Creator4/4
  [Axl1Trq] -> Bus Creator2/1  "Axl1Trq"
  Bus Creator1/1 -> Bus Creator4/1  "Driveshft"
  [DriveshftSpd] -> Power Bus/2(Speed), Bus Creator1/2  "Speed"
  [Axl2Spd] -> Bus Creator3/2  "Axl2Spd"
  Bus Creator4/1 -> Diff/1
  [Axl2Trq] -> Bus Creator3/1  "Axl2Trq"
  [Axl1Spd] -> Bus Creator2/2  "Axl1Spd"
  [DriveshftTrq] -> Bus Creator1/1, Power Bus/1(DriveshftTrq)  "DriveshftTrq"
  DiffPress/1 -> Vector Concatenate1/2, Vector Concatenate1/1, Vector Concatenate1/3, Vector Concatenate1/4
  Vector Concatenate1/1 -> Terminator3/1
  Vector Concatenate/1 -> AxlTrq/1
  Omega/1 -> Demux/1
  Torsional Compliance2/2 -> Vector Concatenate/1, [Axl1Trq]  "T_FL"
  Torsional Compliance1/2 -> Vector Concatenate/2, [Axl2Trq]  "T_FR"
  Constant/1 -> Vector Concatenate/3, Vector Concatenate/4  "T_RR"
  Demux/2 -> Terminator1/1
  Torsional Compliance2/1 -> Limited Slip Differential/2
  Torsional Compliance1/1 -> Limited Slip Differential/3
  Demux/1 -> Demux1/1
  Demux1/2 -> Torsional Compliance1/2
  Limited Slip Differential/4 -> Torsional Compliance1/1, [Axl2Spd]
  DrvShfTrq/1 -> Limited Slip Differential/1, [DriveshftTrq]
  Limited Slip Differential/1 -> Terminator/1
  Demux1/1 -> Torsional Compliance2/2
  Limited Slip Differential/3 -> Torsional Compliance2/1, [Axl1Spd]

== system EV6_LUT_FourWheel_EV6Battery77p4kWh_PowerCorrected/Vehicle Under Test1/Vehicle/Rototest and ORNL Interface/DummyPT ==
  WhlSpeedIn : Inport
  APPToTorque : Lookup_n-D  NumberOfTableDimensions=1  BreakpointsForDimension1=[0 100]  Table=[0 184]  InternalRulePriority=Speed  RndMeth=Simplest
  APPToTorque1 : Lookup_n-D  NumberOfTableDimensions=1  BreakpointsForDimension1=[0 100]  Table=[0 184]  InternalRulePriority=Speed  RndMeth=Simplest
  APP_pct : Constant  Value=0
  BPP_pct : Constant  Value=0
  FDR : Gain  Gain=3.18
  Flip : Gain  Gain=-1
  Gear : Product
  Memory : Memory
  NissanTrans : Lookup_n-D  NumberOfTableDimensions=1  BreakpointsForDimension1=[0 5 10 15 25 34 45 55]  Table=[5.25 3.03 1.95 1.46 1.22 1.00 0.81 0.67]  ExtrapMethod=Clip  InternalRulePriority=Speed  RndMeth=Simplest
  Sum : Sum  Inputs=++|
  WheelRadius : Gain  Gain=0.3235
  kph2mph : Gain  Gain=0.621
  mps2kph : Gain  Gain=3.6
  WheelTorqueOut : Outport
  wires:
  Memory/1 -> WheelTorqueOut/1
  WhlSpeedIn/1 -> WheelRadius/1
  FDR/1 -> Memory/1  "WheelTorqueOut"
  WheelRadius/1 -> mps2kph/1  "Speed_mps"
  Sum/1 -> Gear/1  "TorqueTotal"
  APP_pct/1 -> APPToTorque/1
  Flip/1 -> Sum/2  "BPPTorque"
  APPToTorque1/1 -> Flip/1
  Gear/1 -> FDR/1  "TransTorqueOut"
  NissanTrans/1 -> Gear/2  "Gear"
  BPP_pct/1 -> APPToTorque1/1
  mps2kph/1 -> kph2mph/1  "Speed_kph"
  APPToTorque/1 -> Sum/1  "APPTorque"
  kph2mph/1 -> NissanTrans/1  "Speed_mph"

== system EV6_LUT_FourWheel_EV6Battery77p4kWh_PowerCorrected/Vehicle Under Test1/Vehicle/Rototest and ORNL Interface/Format CM Powertrain Signals ==
  note: Can Bypass with my own brake model
  BrakingTorques : Inport
  RotoWheelSpd : Inport  Port=2
  AxlTrq : Inport  Port=3
  MaxRegen : Inport  Port=4
  Bus Creator1 : BusCreator  Inputs=42
  Bus Selector2 : BusSelector  OutputSignals=Brake IF Trq_WB FL,Brake IF Trq_WB FR,Brake IF Trq_WB RL,Brake IF Trq_WB RR
  BusCreator2 : BusCreator  Inputs=42
  Demux : Demux
  Demux1 : Demux  Outputs=42
      settings: DisplayOption=none
  Demux2 : Demux
  Discrete-Time Integrator{4..7} (4 alike) : DiscreteIntegrator  IntegratorMethod=Integration: Backward Euler  SampleTime=0.001  ICPrevOutput=DiscIntNeverNeededParam  ICPrevScaledInput=DiscIntNeverNeededParam
  Gain{5..8} (4 alike) : Gain  Gain=-1
  Ground{2..5} (4 alike) : Ground
  Ignition : Constant
  Memory{1..4} (4 alike) : Memory
  Operation Error : Constant  Value=4
  Operation State Driving : Constant  Value=4
  Product{1..4} (4 alike) : Product  RndMeth=Zero
  Saturation{1..4} (4 alike) : Saturate  UpperLimit=1  LowerLimit=-1
  Zero{1..5} (5 alike) : Constant  Value=0
  PowerTrainOutIdeal : Outport
  wires:
  Demux2/4 -> Bus Creator1/39  "TrqDrv RR"
  Demux2/3 -> Bus Creator1/32  "TrqDrv RL"
  Demux2/2 -> Bus Creator1/25  "TrqDrv FR"
  Demux2/1 -> Bus Creator1/18  "TrqDrv FL"
  AxlTrq/1 -> Demux2/1
  RotoWheelSpd/1 -> Demux/1
  Saturation3/1 -> Product3/2
  Bus Selector2/4 -> Product4/1  "<Brake IF Trq_WB RR>"
  Product1/1 -> Gain6/1
  Saturation2/1 -> Product2/2
  Bus Creator1/1 -> Demux1/1
  Product4/1 -> Gain8/1
  Demux/1 -> Bus Creator1/16, Discrete-Time Integrator4/1, Memory3/1  "rotv FL"
  Gain7/1 -> Bus Creator1/31
  Bus Selector2/3 -> Product2/1  "<Brake IF Trq_WB RL>"
  Saturation1/1 -> Product1/2
  Memory2/1 -> Saturation2/1
  Ignition/1 -> Bus Creator1/1  "PT Ignition"
  Gain6/1 -> Bus Creator1/24
  Bus Selector2/1 -> Product3/1  "<Brake IF Trq_WB FL>"
  Ground4/1 -> Bus Creator1/6
  Memory1/1 -> Saturation1/1
  Demux/3 -> Bus Creator1/30, Discrete-Time Integrator6/1, Memory2/1  "rotv RL"
  Operation Error/1 -> Bus Creator1/3
  BrakingTorques/1 -> Bus Selector2/1
  Demux1/41 -> BusCreator2/41  "PT IF WRR Trq_BrakeReg"
  Demux1/6 -> BusCreator2/6  "PT IF Trq_Supp2Bdy1 x"
  Zero5/1 -> Bus Creator1/42, Bus Creator1/41, Bus Creator1/40
  Discrete-Time Integrator7/1 -> Bus Creator1/36  "PtT WRR rot"
  Demux/2 -> Bus Creator1/23, Discrete-Time Integrator5/1, Memory1/1  "rotv FR"
  Discrete-Time Integrator4/1 -> Bus Creator1/15  "PT WFL rot"
  Product2/1 -> Gain7/1
  Demux1/20 -> BusCreator2/20  "PT IF WFL Trq_BrakeReg"
  Zero1/1 -> Bus Creator1/8, Bus Creator1/9, Bus Creator1/10, Bus Creator1/11, Bus Creator1/13, Bus Creator1/14, Bus Creator1/12, Bus Creator1/4, Bus Creator1/5
  Zero2/1 -> Bus Creator1/20, Bus Creator1/19
  Demux/4 -> Bus Creator1/37, Discrete-Time Integrator7/1, Memory4/1  "rotv RR"
  Zero3/1 -> Bus Creator1/27, Bus Creator1/26
  Demux1/36 -> BusCreator2/36  "PT IF WRR rot"
  Demux1/32 -> BusCreator2/32  "PT IF WRL Trq_Drive"
  Demux1/31 -> BusCreator2/31  "PT IF WRL Trq_B2W"
  Demux1/37 -> BusCreator2/37  "PT IF WRR rotv"
  Demux1/34 -> BusCreator2/34  "PT IF WRL Trq_BrakeReg"
  Zero4/1 -> Bus Creator1/35, Bus Creator1/34, Bus Creator1/33
  Demux1/39 -> BusCreator2/39  "PT IF WRR Trq_Drive"
  Demux1/35 -> BusCreator2/35  "PT IF WRL Trq_BrakeReg_max"
  Demux1/28 -> BusCreator2/28  "PT IF WFR Trq_BrakeReg_max"
  Demux1/30 -> BusCreator2/30  "PT IF WRL rotv"
  Demux1/33 -> BusCreator2/33  "PT IF WRL Trq_Supp2WC"
  Demux1/29 -> BusCreator2/29  "PT IF WRL rot"
  Demux1/22 -> BusCreator2/22  "PT IF WFR rot"
  Demux1/19 -> BusCreator2/19  "PT IF WFL Trq_Supp2WC"
  Memory3/1 -> Saturation3/1
  Bus Selector2/2 -> Product1/1  "<Brake IF Trq_WB FR>"
  Demux1/15 -> BusCreator2/15  "PT IF WFL rot"
  Demux1/13 -> BusCreator2/13  "PT IF Trq_Supp2BdyEng y"
  Demux1/26 -> BusCreator2/26  "PT IF WFR Trq_Supp2WC"
  Demux1/25 -> BusCreator2/25  "PT IF WFR Trq_Drive"
  Demux1/24 -> BusCreator2/24  "PT IF WFR Trq_B2W"
  Demux1/27 -> BusCreator2/27  "PT IF WFR Trq_BrakeReg"
  Demux1/10 -> BusCreator2/10  "PT IF Trq_Supp2Bdy1B y"
  Memory4/1 -> Saturation4/1
  Demux1/38 -> BusCreator2/38  "PT IF WRR Trq_B2W"
  Demux1/8 -> BusCreator2/8  "PT IF Trq_Supp2Bdy1 z"
  Demux1/18 -> BusCreator2/18  "PT IF WFL Trq_Drive"
  Gain5/1 -> Bus Creator1/17
  Demux1/42 -> BusCreator2/42  "PT IF WRR Trq_BrakeReg_max"
  Discrete-Time Integrator5/1 -> Bus Creator1/22  "PT WFR rot"
  Demux1/7 -> BusCreator2/7  "PT IF Trq_Supp2Bdy1 y"
  Demux1/12 -> BusCreator2/12  "PT IF Trq_Supp2BdyEng x"
  Demux1/11 -> BusCreator2/11  "PT IF Trq_Supp2Bdy1B z"
  Demux1/5 -> BusCreator2/5  "PT IF Engine_rotv"
  Product3/1 -> Gain5/1
  Demux1/17 -> BusCreator2/17  "PT IF WFL Trq_B2W"
  Demux1/4 -> BusCreator2/4  "PT IF GearNo"
  Demux1/14 -> BusCreator2/14  "PT IF DL_iDiff_mean"
  Demux1/23 -> BusCreator2/23  "PT IF WFR rotv"
  Ground2/1 -> Bus Creator1/7
  Demux1/21 -> BusCreator2/21  "PT IF WFL Trq_BrakeReg_max"
  Demux1/16 -> BusCreator2/16  "PT IF WFL rotv"
  Gain8/1 -> Bus Creator1/38
  Operation State Driving/1 -> Bus Creator1/2
  BusCreator2/1 -> PowerTrainOutIdeal/1
  MaxRegen/1 -> Bus Creator1/21, Bus Creator1/28
  Demux1/1 -> BusCreator2/1  "PT IF Ignition"
  Discrete-Time Integrator6/1 -> Bus Creator1/29  "PT WRL rot"
  Demux1/9 -> BusCreator2/9  "PT IF Trq_Supp2Bdy1B x"
  Demux1/40 -> BusCreator2/40  "PT IF WRR Trq_Supp2WC"
  Demux1/2 -> BusCreator2/2  "PT IF OperationState"
  Demux1/3 -> BusCreator2/3  "PT IF OperationError"
  Saturation4/1 -> Product4/2

== system EV6_LUT_FourWheel_EV6Battery77p4kWh_PowerCorrected/Vehicle Under Test1/Vehicle/Rototest and ORNL Interface/From Rototest ==
  Input : Inport
  Bus Creator : BusCreator  Inputs=30
  Bus Selector1 : BusSelector  OutputSignals=ActSpLF_rpm,ActSpRF_rpm,ActSpLR_rpm,ActSpRR_rpm
  Mux1 : Mux
  RotoTestEthRX : Subsystem  AncestorBlock=VSIGenLib/RotoTestEthRX
      mask Display:
      | color('white')
      | disp('RotTestEthTx')
      | port_label('output', 1, 'ID')
      | port_label('output', 2, 'ProtocolVer')
      | port_label('output', 3, 'ActTqLF (Nm)')
      | port_label('output', 4, 'RefRR_NmORrpm')
      | port_label('output', 5, 'ActTempLF (C)')
      | port_label('output', 6, 'ActTqRF (Nm)')
      | port_label('output', 7, 'ActSpRF (rpm)')
      | port_label('output', 8, 'ActTempRF (C)')
      | port_label('output', 9, 'ActTqLR (Nm)')
      | port_label('output', 10, 'ActSpLR (rpm)')
      | port_label('output', 11, 'ActTempLR (C)')
      | port_label('output', 12, 'ActTqRR (Nm)')
      | port_label('output', 13, 'ActSpRR (rpm)')
      | port_label('output', 14, 'ActTempRR (Nm)')
      | port_label('output', 15, 'RefLF (Nm)')
      | port_label('output', 16, 'RefRF (rpm)')
      | port_label('output', 17, 'RefLR (Nm)')
      | port_label('output', 18, 'RefRR (Nm)')
      | port_label('output', 19, 'UnitsStatusLF (enum)')
      | port_label('output', 20, 'UnitsStatusRF (enum)')
      | port_label('output', 21, 'UnitsStatusLR (enum)')
      | port_label('output', 22, 'UnitsStatusRR (enum)')
      | port_label('output', 23, 'WatchdogCnt (int)')
      | port_label('output', 24, 'FaultActive (enum)')
      | port_label('output', 25, 'WarningsActive (enum)')
      | port_label('output', 26, 'SpTqRR (enum)')
      | port_label('output', 27, 'SpTqLR (enum)')
      | port_label('output', 28, 'SpTqRF (enum)')
      | port_label('output', 29, 'SpTqLF (enum)')
      | port_label('output', 30, 'SystemActive (bool)')
  SpdAct : Outport
  AxlTrq : Outport  Port=2
  wires:
  Input/1 -> RotoTestEthRX/1(Input)
  RotoTestEthRX/12(ActTqRR_Nm) -> Bus Creator/12
  RotoTestEthRX/10(ActSpLR_rpm) -> Bus Creator/10
  RotoTestEthRX/13(ActSpRR_rpm) -> Bus Creator/13
  RotoTestEthRX/9(ActTqLR_Nm) -> Bus Creator/9
  RotoTestEthRX/6(ActTqRF_Nm_) -> Bus Creator/6
  RotoTestEthRX/3(ActTqLF_Nm) -> Bus Creator/3
  RotoTestEthRX/14(ActTempRR_Nm) -> Bus Creator/14
  RotoTestEthRX/26(SpTqRR) -> Bus Creator/26
  RotoTestEthRX/27(SpTqLR) -> Bus Creator/27
  RotoTestEthRX/29(SpTqLF) -> Bus Creator/29
  RotoTestEthRX/28(SpTqRF) -> Bus Creator/28
  RotoTestEthRX/1(ID) -> Bus Creator/1
  RotoTestEthRX/11(ActTempLR_C) -> Bus Creator/11
  RotoTestEthRX/21(UnitsStatusLR) -> Bus Creator/21
  RotoTestEthRX/7(ActSpRF_rpm) -> Bus Creator/7
  RotoTestEthRX/2(ProtocolVer) -> Bus Creator/2
  RotoTestEthRX/17(RefLR_Nm) -> Bus Creator/17
  RotoTestEthRX/16(RefRF_rpm) -> Bus Creator/16
  RotoTestEthRX/15(RefLF_Nm) -> Bus Creator/15
  RotoTestEthRX/20(UnitsStatusRF) -> Bus Creator/20
  RotoTestEthRX/30(SystemActive) -> Bus Creator/30
  RotoTestEthRX/5(ActTempLF_C) -> Bus Creator/5
  Bus Selector1/2 -> Mux1/2  "<ActSpRF_rpm>"
  Bus Selector1/1 -> Mux1/1  "<ActSpLF_rpm>"
  RotoTestEthRX/25(WarningsActive) -> Bus Creator/25
  Bus Selector1/3 -> Mux1/3  "<ActSpLR_rpm>"
  RotoTestEthRX/22(UnitsStatusRR) -> Bus Creator/22
  RotoTestEthRX/24(FaultActive) -> Bus Creator/24
  Bus Selector1/4 -> Mux1/4  "<ActSpRR_rpm>"
  Bus Creator/1 -> Bus Selector1/1, AxlTrq/1
  RotoTestEthRX/4(ActSpLF_rpm) -> Bus Creator/4
  RotoTestEthRX/19(UnitsStatusLF) -> Bus Creator/19
  Mux1/1 -> SpdAct/1
  RotoTestEthRX/18(RefRR_Nm) -> Bus Creator/18
  RotoTestEthRX/23(WatchdogCnt) -> Bus Creator/23
  RotoTestEthRX/8(ActTempRF_C) -> Bus Creator/8

== system EV6_LUT_FourWheel_EV6Battery77p4kWh_PowerCorrected/Vehicle Under Test1/Vehicle/Rototest and ORNL Interface/Get Wheel Spd Cmd Based on Wheel Dynamics ==
  BrakingTorques : Inport
  Trq_T2W : Inport  Port=2
  AxlTrq : Inport  Port=3
  MaxRegen : Inport  Port=4
  FxIn : Inport  Port=5
  Saturation : Saturate  UpperLimit=100  LowerLimit=0
  Saturation1 : Saturate  UpperLimit=300  LowerLimit=-300
  Scope : Scope
  WheelSpdCmd : Subsystem
  Whl Dynamics & Format CM Powertrain Signal : Subsystem
  WhlSpdCmd : Outport
  wires:
  Saturation/1 -> WhlSpdCmd/1
  [SimOmega] -> Saturation/1, Scope/1
  FxIn/1 -> Whl Dynamics & Format CM Powertrain Signal/5(FxIn)
  AxlTrq/1 -> Whl Dynamics & Format CM Powertrain Signal/3(AxlTrq)
  MaxRegen/1 -> Whl Dynamics & Format CM Powertrain Signal/4(MaxRegen)
  Trq_T2W/1 -> Whl Dynamics & Format CM Powertrain Signal/2(Trq_T2W)
  BrakingTorques/1 -> Whl Dynamics & Format CM Powertrain Signal/1(BrakingTorques)
  Whl Dynamics & Format CM Powertrain Signal/1(PowerTrainOutIdeal) -> WheelSpdCmd/1(In1)
